simulink model "fft_direct_test"  (Simulink 7.2)
settings: Solver=VariableStepDiscrete  StartTime=0.0  StopTime=250  RelTol=1e-3
libraries: xbsIndex_r4 x249, casper_library_misc x24, simulink x1
(part 2 of 3)

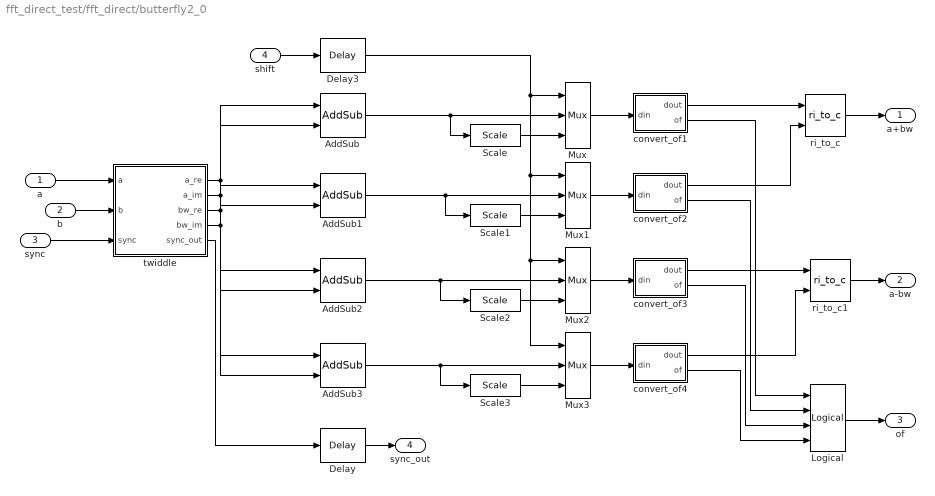
== system fft_direct_test/fft_direct/butterfly2_0 ==
  a : Inport  OutDataType=sfix(16)  OutScaling=2^0
  b : Inport  Port=2  OutDataType=sfix(16)  OutScaling=2^0
  sync : Inport  Port=3  OutDataType=sfix(16)  OutScaling=2^0
  shift : Inport  Port=4  OutDataType=sfix(16)  OutScaling=2^0
  AddSub : xbsIndex_r4/AddSub  mode=Addition  use_carryin=off  use_carryout=off  en=off  latency=add_latency  precision=Full  arith_type=Unsigned  n_bits=8  bin_pt=2  quantization=Truncate  overflow=Wrap  dbl_ovrd=off  use_behavioral_HDL=on  hw_selection=DSP48  pipelined=on  use_rpm=on  block_type=addsub
      settings: xl_area=[0, 0, 0, 0, 0, 0, 0]  block_version=9.1.01
  AddSub1 : xbsIndex_r4/AddSub  mode=Addition  use_carryin=off  use_carryout=off  en=off  latency=add_latency  precision=Full  arith_type=Unsigned  n_bits=8  bin_pt=2  quantization=Truncate  overflow=Wrap  dbl_ovrd=off  use_behavioral_HDL=on  hw_selection=DSP48  pipelined=on  use_rpm=on  block_type=addsub
      settings: xl_area=[0, 0, 0, 0, 0, 0, 0]  block_version=9.1.01
  AddSub2 : xbsIndex_r4/AddSub  mode=Subtraction  use_carryin=off  use_carryout=off  en=off  latency=add_latency  precision=Full  arith_type=Unsigned  n_bits=8  bin_pt=2  quantization=Truncate  overflow=Wrap  dbl_ovrd=off  use_behavioral_HDL=on  hw_selection=DSP48  pipelined=on  use_rpm=on  block_type=addsub
      settings: xl_area=[0, 0, 0, 0, 0, 0, 0]  block_version=9.1.01
  AddSub3 : xbsIndex_r4/AddSub  mode=Subtraction  use_carryin=off  use_carryout=off  en=off  latency=add_latency  precision=Full  arith_type=Unsigned  n_bits=8  bin_pt=2  quantization=Truncate  overflow=Wrap  dbl_ovrd=off  use_behavioral_HDL=on  hw_selection=DSP48  pipelined=on  use_rpm=on  block_type=addsub
      settings: xl_area=[0, 0, 0, 0, 0, 0, 0]  block_version=9.1.01
  Delay : xbsIndex_r4/Delay  en=off  latency=add_latency + conv_latency + 1  dbl_ovrd=off  reg_retiming=on  block_type=delay
      settings: xl_area=[0, 0, 0, 0, 0, 0, 0]  block_version=9.1.01
  Delay3 : xbsIndex_r4/Delay  en=off  latency=add_latency  dbl_ovrd=off  reg_retiming=off  block_type=delay
      settings: xl_area=[0, 0, 0, 0, 0, 0, 0]  block_version=9.1.01
  Logical : xbsIndex_r4/Logical  logical_function=OR  inputs=4  en=off  latency=0  precision=Full  arith_type=Unsigned  n_bits=16  bin_pt=0  align_bp=on  dbl_ovrd=off  block_type=logical
      settings: block_version=10.1.1
  Mux{,1..3} (4 alike) : xbsIndex_r4/Mux  inputs=2  en=off  latency=1  precision=Full  arith_type="Signed  (2's comp)"  n_bits=8  bin_pt=2  quantization=Truncate  overflow=Wrap  dbl_ovrd=off  block_type=mux
      settings: xl_area=[0, 0, 0, 0, 0, 0, 0]  block_version=9.1.01
  Scale{,1..3} (4 alike) : xbsIndex_r4/Scale  scale_factor=-1  dbl_ovrd=off  block_type=scale
      settings: infoedit=Scales input by a power of two by adjusting the binary point position.<P><P>Hardware notes: In hardware this block costs nothing.  block_version=9.1.01
  convert_of1 : Subsystem  AncestorBlock=casper_library_misc/convert_of  mask(convert_of){bit_width_i=14, binary_point_i=12, bit_width_o=12, binary_point_o=11, latency=2, overflow=Saturate, quantization=Truncate}
      mask prompts: bit_width_i "Bit Width In"; binary_point_i "Binary Point In"; bit_width_o "Bit Width Out"; binary_point_o "Binary Point Out"; overflow "Overflow Behaviour"; quantization "Quantization Behaviour"
      mask help:
      | Converts from one 2's complement bit-width
      | and/or binary point position to another.
      | Includes underflow/overflow indicator.
      mask init: same as fft_direct_test/fft_direct/butterfly1_0/convert_of1
      settings: AttributesFormatString=[14,12]->[12,11]
      mask StyleString: edit,edit,edit,edit,edit,popup(Wrap|Saturate|Error),popup(Truncate|Round  (unbiased: +/- Inf)|Round  (unbiased: even values))
  convert_of2 : Subsystem  AncestorBlock=casper_library_misc/convert_of  mask(convert_of){bit_width_i=14, binary_point_i=12, bit_width_o=12, binary_point_o=11, latency=2, overflow=Saturate, quantization=Truncate}
      mask prompts: bit_width_i "Bit Width In"; binary_point_i "Binary Point In"; bit_width_o "Bit Width Out"; binary_point_o "Binary Point Out"; overflow "Overflow Behaviour"; quantization "Quantization Behaviour"
      mask help:
      | Converts from one 2's complement bit-width
      | and/or binary point position to another.
      | Includes underflow/overflow indicator.
      mask init: same as fft_direct_test/fft_direct/butterfly1_0/convert_of1
      settings: AttributesFormatString=[14,12]->[12,11]
      mask StyleString: edit,edit,edit,edit,edit,popup(Wrap|Saturate|Error),popup(Truncate|Round  (unbiased: +/- Inf)|Round  (unbiased: even values))
  convert_of3 : Subsystem  AncestorBlock=casper_library_misc/convert_of  mask(convert_of){bit_width_i=14, binary_point_i=12, bit_width_o=12, binary_point_o=11, latency=2, overflow=Saturate, quantization=Truncate}
      mask prompts: bit_width_i "Bit Width In"; binary_point_i "Binary Point In"; bit_width_o "Bit Width Out"; binary_point_o "Binary Point Out"; overflow "Overflow Behaviour"; quantization "Quantization Behaviour"
      mask help:
      | Converts from one 2's complement bit-width
      | and/or binary point position to another.
      | Includes underflow/overflow indicator.
      mask init: same as fft_direct_test/fft_direct/butterfly1_0/convert_of1
      settings: AttributesFormatString=[14,12]->[12,11]
      mask StyleString: edit,edit,edit,edit,edit,popup(Wrap|Saturate|Error),popup(Truncate|Round  (unbiased: +/- Inf)|Round  (unbiased: even values))
  convert_of4 : Subsystem  AncestorBlock=casper_library_misc/convert_of  mask(convert_of){bit_width_i=14, binary_point_i=12, bit_width_o=12, binary_point_o=11, latency=2, overflow=Saturate, quantization=Truncate}
      mask prompts: bit_width_i "Bit Width In"; binary_point_i "Binary Point In"; bit_width_o "Bit Width Out"; binary_point_o "Binary Point Out"; overflow "Overflow Behaviour"; quantization "Quantization Behaviour"
      mask help:
      | Converts from one 2's complement bit-width
      | and/or binary point position to another.
      | Includes underflow/overflow indicator.
      mask init: same as fft_direct_test/fft_direct/butterfly1_0/convert_of1
      settings: AttributesFormatString=[14,12]->[12,11]
      mask StyleString: edit,edit,edit,edit,edit,popup(Wrap|Saturate|Error),popup(Truncate|Round  (unbiased: +/- Inf)|Round  (unbiased: even values))
  ri_to_c : casper_library_misc/ri_to_c  SystemSampleTime=-1
  ri_to_c1 : casper_library_misc/ri_to_c  SystemSampleTime=-1
  twiddle : Subsystem  AncestorBlock=casper_library_ffts_twiddle/twiddle_coeff_0  mask(twiddle_coeff_0){FFTSize=2, input_bit_width=12, add_latency=1, mult_latency=2, bram_latency=1, conv_latency=2, opt_target=multipliers}
      mask prompts: FFTSize "FFT Size (2^?)"; input_bit_width "Input Bit Width"; add_latency "Add Latency"; mult_latency "Mult Latency"; bram_latency "BRAM Latency"; conv_latency "Convert latency"; opt_target "Use less"
      mask help:
      | Used in FFT library. Used when coefficients
      | are 2^0 (just pass data through) but latency
      | must be the same as for a full twiddle.
      mask init: same as fft_direct_test/fft_direct/butterfly1_0/twiddle
      mask StyleString: edit,edit,edit,edit,edit,edit,popup(logic|multipliers)
  a+bw : Outport  OutDataType=sfix(16)  OutScaling=2^0
  a-bw : Outport  Port=2  OutDataType=sfix(16)  OutScaling=2^0
  of : Outport  Port=3  OutDataType=sfix(16)  OutScaling=2^0
  sync_out : Outport  Port=4  OutDataType=sfix(16)  OutScaling=2^0
  wires:
  convert_of4/2(of) -> Logical/4
  convert_of3/2(of) -> Logical/3
  convert_of2/2(of) -> Logical/2
  convert_of1/2(of) -> Logical/1
  convert_of4/1(dout) -> ri_to_c1/2
  Mux3/1 -> convert_of4/1(din)
  AddSub3/1 -> Scale3/1, Mux3/2
  Scale3/1 -> Mux3/3
  convert_of3/1(dout) -> ri_to_c1/1
  Mux2/1 -> convert_of3/1(din)
  AddSub2/1 -> Scale2/1, Mux2/2
  Scale2/1 -> Mux2/3
  convert_of2/1(dout) -> ri_to_c/2
  Mux1/1 -> convert_of2/1(din)
  AddSub1/1 -> Scale1/1, Mux1/2
  Scale1/1 -> Mux1/3
  convert_of1/1(dout) -> ri_to_c/1
  Mux/1 -> convert_of1/1(din)
  twiddle/4(bw_im) -> AddSub3/2, AddSub1/2
  twiddle/3(bw_re) -> AddSub2/2, AddSub/2
  twiddle/2(a_im) -> AddSub3/1, AddSub1/1
  twiddle/1(a_re) -> AddSub2/1, AddSub/1
  sync/1 -> twiddle/3(sync)
  b/1 -> twiddle/2(b)
  a/1 -> twiddle/1(a)
  ri_to_c/1 -> a+bw/1
  ri_to_c1/1 -> a-bw/1
  Delay/1 -> sync_out/1
  AddSub/1 -> Mux/2, Scale/1
  shift/1 -> Delay3/1
  Scale/1 -> Mux/3
  Delay3/1 -> Mux3/1, Mux2/1, Mux1/1, Mux/1
  Logical/1 -> of/1
  twiddle/5(sync_out) -> Delay/1

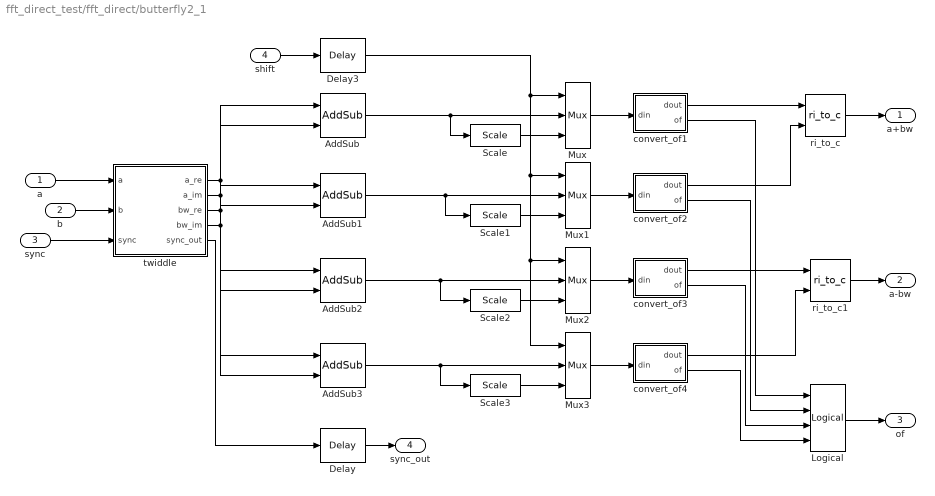
== system fft_direct_test/fft_direct/butterfly2_1 ==
  a : Inport  OutDataType=sfix(16)  OutScaling=2^0
  b : Inport  Port=2  OutDataType=sfix(16)  OutScaling=2^0
  sync : Inport  Port=3  OutDataType=sfix(16)  OutScaling=2^0
  shift : Inport  Port=4  OutDataType=sfix(16)  OutScaling=2^0
  AddSub : xbsIndex_r4/AddSub  mode=Addition  use_carryin=off  use_carryout=off  en=off  latency=add_latency  precision=Full  arith_type=Unsigned  n_bits=8  bin_pt=2  quantization=Truncate  overflow=Wrap  dbl_ovrd=off  use_behavioral_HDL=on  hw_selection=DSP48  pipelined=on  use_rpm=on  block_type=addsub
      settings: xl_area=[0, 0, 0, 0, 0, 0, 0]  block_version=9.1.01
  AddSub1 : xbsIndex_r4/AddSub  mode=Addition  use_carryin=off  use_carryout=off  en=off  latency=add_latency  precision=Full  arith_type=Unsigned  n_bits=8  bin_pt=2  quantization=Truncate  overflow=Wrap  dbl_ovrd=off  use_behavioral_HDL=on  hw_selection=DSP48  pipelined=on  use_rpm=on  block_type=addsub
      settings: xl_area=[0, 0, 0, 0, 0, 0, 0]  block_version=9.1.01
  AddSub2 : xbsIndex_r4/AddSub  mode=Subtraction  use_carryin=off  use_carryout=off  en=off  latency=add_latency  precision=Full  arith_type=Unsigned  n_bits=8  bin_pt=2  quantization=Truncate  overflow=Wrap  dbl_ovrd=off  use_behavioral_HDL=on  hw_selection=DSP48  pipelined=on  use_rpm=on  block_type=addsub
      settings: xl_area=[0, 0, 0, 0, 0, 0, 0]  block_version=9.1.01
  AddSub3 : xbsIndex_r4/AddSub  mode=Subtraction  use_carryin=off  use_carryout=off  en=off  latency=add_latency  precision=Full  arith_type=Unsigned  n_bits=8  bin_pt=2  quantization=Truncate  overflow=Wrap  dbl_ovrd=off  use_behavioral_HDL=on  hw_selection=DSP48  pipelined=on  use_rpm=on  block_type=addsub
      settings: xl_area=[0, 0, 0, 0, 0, 0, 0]  block_version=9.1.01
  Delay : xbsIndex_r4/Delay  en=off  latency=add_latency + conv_latency + 1  dbl_ovrd=off  reg_retiming=on  block_type=delay
      settings: xl_area=[0, 0, 0, 0, 0, 0, 0]  block_version=9.1.01
  Delay3 : xbsIndex_r4/Delay  en=off  latency=add_latency  dbl_ovrd=off  reg_retiming=off  block_type=delay
      settings: xl_area=[0, 0, 0, 0, 0, 0, 0]  block_version=9.1.01
  Logical : xbsIndex_r4/Logical  logical_function=OR  inputs=4  en=off  latency=0  precision=Full  arith_type=Unsigned  n_bits=16  bin_pt=0  align_bp=on  dbl_ovrd=off  block_type=logical
      settings: block_version=10.1.1
  Mux{,1..3} (4 alike) : xbsIndex_r4/Mux  inputs=2  en=off  latency=1  precision=Full  arith_type="Signed  (2's comp)"  n_bits=8  bin_pt=2  quantization=Truncate  overflow=Wrap  dbl_ovrd=off  block_type=mux
      settings: xl_area=[0, 0, 0, 0, 0, 0, 0]  block_version=9.1.01
  Scale{,1..3} (4 alike) : xbsIndex_r4/Scale  scale_factor=-1  dbl_ovrd=off  block_type=scale
      settings: infoedit=Scales input by a power of two by adjusting the binary point position.<P><P>Hardware notes: In hardware this block costs nothing.  block_version=9.1.01
  convert_of1 : Subsystem  AncestorBlock=casper_library_misc/convert_of  mask(convert_of){bit_width_i=14, binary_point_i=12, bit_width_o=12, binary_point_o=11, latency=2, overflow=Saturate, quantization=Truncate}
      mask prompts: bit_width_i "Bit Width In"; binary_point_i "Binary Point In"; bit_width_o "Bit Width Out"; binary_point_o "Binary Point Out"; overflow "Overflow Behaviour"; quantization "Quantization Behaviour"
      mask help:
      | Converts from one 2's complement bit-width
      | and/or binary point position to another.
      | Includes underflow/overflow indicator.
      mask init: same as fft_direct_test/fft_direct/butterfly1_0/convert_of1
      settings: AttributesFormatString=[14,12]->[12,11]
      mask StyleString: edit,edit,edit,edit,edit,popup(Wrap|Saturate|Error),popup(Truncate|Round  (unbiased: +/- Inf)|Round  (unbiased: even values))
  convert_of2 : Subsystem  AncestorBlock=casper_library_misc/convert_of  mask(convert_of){bit_width_i=14, binary_point_i=12, bit_width_o=12, binary_point_o=11, latency=2, overflow=Saturate, quantization=Truncate}
      mask prompts: bit_width_i "Bit Width In"; binary_point_i "Binary Point In"; bit_width_o "Bit Width Out"; binary_point_o "Binary Point Out"; overflow "Overflow Behaviour"; quantization "Quantization Behaviour"
      mask help:
      | Converts from one 2's complement bit-width
      | and/or binary point position to another.
      | Includes underflow/overflow indicator.
      mask init: same as fft_direct_test/fft_direct/butterfly1_0/convert_of1
      settings: AttributesFormatString=[14,12]->[12,11]
      mask StyleString: edit,edit,edit,edit,edit,popup(Wrap|Saturate|Error),popup(Truncate|Round  (unbiased: +/- Inf)|Round  (unbiased: even values))
  convert_of3 : Subsystem  AncestorBlock=casper_library_misc/convert_of  mask(convert_of){bit_width_i=14, binary_point_i=12, bit_width_o=12, binary_point_o=11, latency=2, overflow=Saturate, quantization=Truncate}
      mask prompts: bit_width_i "Bit Width In"; binary_point_i "Binary Point In"; bit_width_o "Bit Width Out"; binary_point_o "Binary Point Out"; overflow "Overflow Behaviour"; quantization "Quantization Behaviour"
      mask help:
      | Converts from one 2's complement bit-width
      | and/or binary point position to another.
      | Includes underflow/overflow indicator.
      mask init: same as fft_direct_test/fft_direct/butterfly1_0/convert_of1
      settings: AttributesFormatString=[14,12]->[12,11]
      mask StyleString: edit,edit,edit,edit,edit,popup(Wrap|Saturate|Error),popup(Truncate|Round  (unbiased: +/- Inf)|Round  (unbiased: even values))
  convert_of4 : Subsystem  AncestorBlock=casper_library_misc/convert_of  mask(convert_of){bit_width_i=14, binary_point_i=12, bit_width_o=12, binary_point_o=11, latency=2, overflow=Saturate, quantization=Truncate}
      mask prompts: bit_width_i "Bit Width In"; binary_point_i "Binary Point In"; bit_width_o "Bit Width Out"; binary_point_o "Binary Point Out"; overflow "Overflow Behaviour"; quantization "Quantization Behaviour"
      mask help:
      | Converts from one 2's complement bit-width
      | and/or binary point position to another.
      | Includes underflow/overflow indicator.
      mask init: same as fft_direct_test/fft_direct/butterfly1_0/convert_of1
      settings: AttributesFormatString=[14,12]->[12,11]
      mask StyleString: edit,edit,edit,edit,edit,popup(Wrap|Saturate|Error),popup(Truncate|Round  (unbiased: +/- Inf)|Round  (unbiased: even values))
  ri_to_c : casper_library_misc/ri_to_c  SystemSampleTime=-1
  ri_to_c1 : casper_library_misc/ri_to_c  SystemSampleTime=-1
  twiddle : Subsystem  AncestorBlock=casper_library_ffts_twiddle/twiddle_coeff_1  mask(twiddle_coeff_1){FFTSize=2, input_bit_width=12, add_latency=1, mult_latency=2, bram_latency=1, conv_latency=2, opt_target=multipliers}
      mask prompts: FFTSize "FFT Size (2^?)"; input_bit_width "Input Bit Width"; add_latency "Add Latency"; mult_latency "Mult Latency"; bram_latency "BRAM Latency"; conv_latency "Convert latency"; opt_target "Use less"
      mask help:
      | Used in FFT library. Used when result of
      | coeff*(a+jb)=b-ja
      mask init:
      | set_param(gcb,'LinkStatus','inactive');
      | if(strcmp(opt_target, 'logic')), 
      |     latency = 'mult_latency+add_latency+bram_latency+conv_latency';
      | else,
      |     latency = 'mult_latency+add_latency*2+bram_latency+conv_latency';
      | end
      | set_param([gcb,'/delay0'], 'latency', latency);
      | set_param([gcb,'/delay1'], 'latency', latency);
      | set_param([gcb,'/delay2'], 'latency', latency);
      | set_param([gcb,'/delay3'], 'latency', latency);
      | set_param([gcb,'/negate'], 'latency', latency);
      mask StyleString: edit,edit,edit,edit,edit,edit,popup(logic|multipliers)
  a+bw : Outport  OutDataType=sfix(16)  OutScaling=2^0
  a-bw : Outport  Port=2  OutDataType=sfix(16)  OutScaling=2^0
  of : Outport  Port=3  OutDataType=sfix(16)  OutScaling=2^0
  sync_out : Outport  Port=4  OutDataType=sfix(16)  OutScaling=2^0
  wires:
  convert_of4/2(of) -> Logical/4
  convert_of3/2(of) -> Logical/3
  convert_of2/2(of) -> Logical/2
  convert_of1/2(of) -> Logical/1
  convert_of4/1(dout) -> ri_to_c1/2
  Mux3/1 -> convert_of4/1(din)
  AddSub3/1 -> Scale3/1, Mux3/2
  Scale3/1 -> Mux3/3
  convert_of3/1(dout) -> ri_to_c1/1
  Mux2/1 -> convert_of3/1(din)
  AddSub2/1 -> Scale2/1, Mux2/2
  Scale2/1 -> Mux2/3
  convert_of2/1(dout) -> ri_to_c/2
  Mux1/1 -> convert_of2/1(din)
  AddSub1/1 -> Scale1/1, Mux1/2
  Scale1/1 -> Mux1/3
  convert_of1/1(dout) -> ri_to_c/1
  Mux/1 -> convert_of1/1(din)
  twiddle/4(bw_im) -> AddSub3/2, AddSub1/2
  twiddle/3(bw_re) -> AddSub2/2, AddSub/2
  twiddle/2(a_im) -> AddSub3/1, AddSub1/1
  twiddle/1(a_re) -> AddSub2/1, AddSub/1
  sync/1 -> twiddle/3(sync)
  b/1 -> twiddle/2(b)
  a/1 -> twiddle/1(a)
  ri_to_c/1 -> a+bw/1
  ri_to_c1/1 -> a-bw/1
  Delay/1 -> sync_out/1
  AddSub/1 -> Mux/2, Scale/1
  shift/1 -> Delay3/1
  Scale/1 -> Mux/3
  Delay3/1 -> Mux3/1, Mux2/1, Mux1/1, Mux/1
  Logical/1 -> of/1
  twiddle/5(sync_out) -> Delay/1

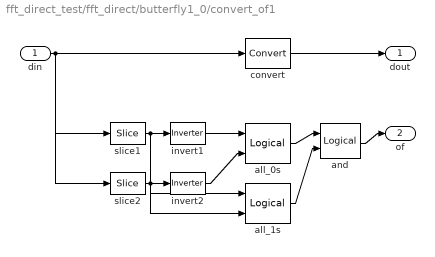
== system fft_direct_test/fft_direct/butterfly1_0/convert_of1 ==
  din : Inport  OutDataType=sfix(16)  OutScaling=2^0
  all_0s : xbsIndex_r4/Logical  logical_function=NAND  inputs=2  en=off  latency=latency  precision=Full  arith_type=Unsigned  n_bits=16  bin_pt=0  align_bp=on  dbl_ovrd=off  block_type=logical
  all_1s : xbsIndex_r4/Logical  logical_function=NAND  inputs=2  en=off  latency=latency  precision=Full  arith_type=Unsigned  n_bits=16  bin_pt=0  align_bp=on  dbl_ovrd=off  block_type=logical
  and : xbsIndex_r4/Logical  logical_function=AND  inputs=2  en=off  latency=0  precision=Full  arith_type=Unsigned  n_bits=16  bin_pt=0  align_bp=on  dbl_ovrd=off  block_type=logical
  convert : xbsIndex_r4/Convert  arith_type="Signed  (2's comp)"  n_bits=bit_width_o  bin_pt=binary_point_o  quantization=Truncate  overflow=Saturate  latency=latency  dbl_ovrd=off  pipeline=on  block_type=convert
      settings: block_version=10.1.1
  invert1 : xbsIndex_r4/Inverter  en=off  latency=0  dbl_ovrd=off  block_type=inv
  invert2 : xbsIndex_r4/Inverter  en=off  latency=0  dbl_ovrd=off  block_type=inv
  slice1 : xbsIndex_r4/Slice  nbits=1  boolean_output=on  mode=Upper Bit Location + Width  bit1=0  base1=MSB of Input  bit0=0  base0=LSB of Input  dbl_ovrd=off  block_type=slice
      settings: infoedit="Extracts a given range of bits from each input sample and presents it at the output.  The output type is ordinarily unsigned with binary point at zero, but can be Boolean when the slice is one bit wide.<P><P>Hardware notes: In hardware this block costs nothing."  block_version=10.1.1
  slice2 : xbsIndex_r4/Slice  nbits=1  boolean_output=on  mode=Upper Bit Location + Width  bit1=-1  base1=MSB of Input  bit0=0  base0=LSB of Input  dbl_ovrd=off  block_type=slice
      settings: infoedit="Extracts a given range of bits from each input sample and presents it at the output.  The output type is ordinarily unsigned with binary point at zero, but can be Boolean when the slice is one bit wide.<P><P>Hardware notes: In hardware this block costs nothing."  block_version=10.1.1
  dout : Outport
  of : Outport  Port=2
  wires:
  din/1 -> convert/1, slice1/1, slice2/1
  convert/1 -> dout/1
  slice1/1 -> all_1s/1, invert1/1
  invert1/1 -> all_0s/1
  slice2/1 -> all_1s/2, invert2/1
  invert2/1 -> all_0s/2
  all_0s/1 -> and/1
  all_1s/1 -> and/2
  and/1 -> of/1

== system fft_direct_test/fft_direct/butterfly1_0/convert_of2 ==
  din : Inport  OutDataType=sfix(16)  OutScaling=2^0
  all_0s : xbsIndex_r4/Logical  logical_function=NAND  inputs=2  en=off  latency=latency  precision=Full  arith_type=Unsigned  n_bits=16  bin_pt=0  align_bp=on  dbl_ovrd=off  block_type=logical
  all_1s : xbsIndex_r4/Logical  logical_function=NAND  inputs=2  en=off  latency=latency  precision=Full  arith_type=Unsigned  n_bits=16  bin_pt=0  align_bp=on  dbl_ovrd=off  block_type=logical
  and : xbsIndex_r4/Logical  logical_function=AND  inputs=2  en=off  latency=0  precision=Full  arith_type=Unsigned  n_bits=16  bin_pt=0  align_bp=on  dbl_ovrd=off  block_type=logical
  convert : xbsIndex_r4/Convert  arith_type="Signed  (2's comp)"  n_bits=bit_width_o  bin_pt=binary_point_o  quantization=Truncate  overflow=Saturate  latency=latency  dbl_ovrd=off  pipeline=on  block_type=convert
      settings: block_version=10.1.1
  invert1 : xbsIndex_r4/Inverter  en=off  latency=0  dbl_ovrd=off  block_type=inv
  invert2 : xbsIndex_r4/Inverter  en=off  latency=0  dbl_ovrd=off  block_type=inv
  slice1 : xbsIndex_r4/Slice  nbits=1  boolean_output=on  mode=Upper Bit Location + Width  bit1=0  base1=MSB of Input  bit0=0  base0=LSB of Input  dbl_ovrd=off  block_type=slice
      settings: infoedit="Extracts a given range of bits from each input sample and presents it at the output.  The output type is ordinarily unsigned with binary point at zero, but can be Boolean when the slice is one bit wide.<P><P>Hardware notes: In hardware this block costs nothing."  block_version=10.1.1
  slice2 : xbsIndex_r4/Slice  nbits=1  boolean_output=on  mode=Upper Bit Location + Width  bit1=-1  base1=MSB of Input  bit0=0  base0=LSB of Input  dbl_ovrd=off  block_type=slice
      settings: infoedit="Extracts a given range of bits from each input sample and presents it at the output.  The output type is ordinarily unsigned with binary point at zero, but can be Boolean when the slice is one bit wide.<P><P>Hardware notes: In hardware this block costs nothing."  block_version=10.1.1
  dout : Outport
  of : Outport  Port=2
  wires:
  din/1 -> convert/1, slice1/1, slice2/1
  convert/1 -> dout/1
  slice1/1 -> all_1s/1, invert1/1
  invert1/1 -> all_0s/1
  slice2/1 -> all_1s/2, invert2/1
  invert2/1 -> all_0s/2
  all_0s/1 -> and/1
  all_1s/1 -> and/2
  and/1 -> of/1

== system fft_direct_test/fft_direct/butterfly1_0/convert_of3 ==
  din : Inport  OutDataType=sfix(16)  OutScaling=2^0
  all_0s : xbsIndex_r4/Logical  logical_function=NAND  inputs=2  en=off  latency=latency  precision=Full  arith_type=Unsigned  n_bits=16  bin_pt=0  align_bp=on  dbl_ovrd=off  block_type=logical
  all_1s : xbsIndex_r4/Logical  logical_function=NAND  inputs=2  en=off  latency=latency  precision=Full  arith_type=Unsigned  n_bits=16  bin_pt=0  align_bp=on  dbl_ovrd=off  block_type=logical
  and : xbsIndex_r4/Logical  logical_function=AND  inputs=2  en=off  latency=0  precision=Full  arith_type=Unsigned  n_bits=16  bin_pt=0  align_bp=on  dbl_ovrd=off  block_type=logical
  convert : xbsIndex_r4/Convert  arith_type="Signed  (2's comp)"  n_bits=bit_width_o  bin_pt=binary_point_o  quantization=Truncate  overflow=Saturate  latency=latency  dbl_ovrd=off  pipeline=on  block_type=convert
      settings: block_version=10.1.1
  invert1 : xbsIndex_r4/Inverter  en=off  latency=0  dbl_ovrd=off  block_type=inv
  invert2 : xbsIndex_r4/Inverter  en=off  latency=0  dbl_ovrd=off  block_type=inv
  slice1 : xbsIndex_r4/Slice  nbits=1  boolean_output=on  mode=Upper Bit Location + Width  bit1=0  base1=MSB of Input  bit0=0  base0=LSB of Input  dbl_ovrd=off  block_type=slice
      settings: infoedit="Extracts a given range of bits from each input sample and presents it at the output.  The output type is ordinarily unsigned with binary point at zero, but can be Boolean when the slice is one bit wide.<P><P>Hardware notes: In hardware this block costs nothing."  block_version=10.1.1
  slice2 : xbsIndex_r4/Slice  nbits=1  boolean_output=on  mode=Upper Bit Location + Width  bit1=-1  base1=MSB of Input  bit0=0  base0=LSB of Input  dbl_ovrd=off  block_type=slice
      settings: infoedit="Extracts a given range of bits from each input sample and presents it at the output.  The output type is ordinarily unsigned with binary point at zero, but can be Boolean when the slice is one bit wide.<P><P>Hardware notes: In hardware this block costs nothing."  block_version=10.1.1
  dout : Outport
  of : Outport  Port=2
  wires:
  din/1 -> convert/1, slice1/1, slice2/1
  convert/1 -> dout/1
  slice1/1 -> all_1s/1, invert1/1
  invert1/1 -> all_0s/1
  slice2/1 -> all_1s/2, invert2/1
  invert2/1 -> all_0s/2
  all_0s/1 -> and/1
  all_1s/1 -> and/2
  and/1 -> of/1

== system fft_direct_test/fft_direct/butterfly1_0/convert_of4 ==
  din : Inport  OutDataType=sfix(16)  OutScaling=2^0
  all_0s : xbsIndex_r4/Logical  logical_function=NAND  inputs=2  en=off  latency=latency  precision=Full  arith_type=Unsigned  n_bits=16  bin_pt=0  align_bp=on  dbl_ovrd=off  block_type=logical
  all_1s : xbsIndex_r4/Logical  logical_function=NAND  inputs=2  en=off  latency=latency  precision=Full  arith_type=Unsigned  n_bits=16  bin_pt=0  align_bp=on  dbl_ovrd=off  block_type=logical
  and : xbsIndex_r4/Logical  logical_function=AND  inputs=2  en=off  latency=0  precision=Full  arith_type=Unsigned  n_bits=16  bin_pt=0  align_bp=on  dbl_ovrd=off  block_type=logical
  convert : xbsIndex_r4/Convert  arith_type="Signed  (2's comp)"  n_bits=bit_width_o  bin_pt=binary_point_o  quantization=Truncate  overflow=Saturate  latency=latency  dbl_ovrd=off  pipeline=on  block_type=convert
      settings: block_version=10.1.1
  invert1 : xbsIndex_r4/Inverter  en=off  latency=0  dbl_ovrd=off  block_type=inv
  invert2 : xbsIndex_r4/Inverter  en=off  latency=0  dbl_ovrd=off  block_type=inv
  slice1 : xbsIndex_r4/Slice  nbits=1  boolean_output=on  mode=Upper Bit Location + Width  bit1=0  base1=MSB of Input  bit0=0  base0=LSB of Input  dbl_ovrd=off  block_type=slice
      settings: infoedit="Extracts a given range of bits from each input sample and presents it at the output.  The output type is ordinarily unsigned with binary point at zero, but can be Boolean when the slice is one bit wide.<P><P>Hardware notes: In hardware this block costs nothing."  block_version=10.1.1
  slice2 : xbsIndex_r4/Slice  nbits=1  boolean_output=on  mode=Upper Bit Location + Width  bit1=-1  base1=MSB of Input  bit0=0  base0=LSB of Input  dbl_ovrd=off  block_type=slice
      settings: infoedit="Extracts a given range of bits from each input sample and presents it at the output.  The output type is ordinarily unsigned with binary point at zero, but can be Boolean when the slice is one bit wide.<P><P>Hardware notes: In hardware this block costs nothing."  block_version=10.1.1
  dout : Outport
  of : Outport  Port=2
  wires:
  din/1 -> convert/1, slice1/1, slice2/1
  convert/1 -> dout/1
  slice1/1 -> all_1s/1, invert1/1
  invert1/1 -> all_0s/1
  slice2/1 -> all_1s/2, invert2/1
  invert2/1 -> all_0s/2
  all_0s/1 -> and/1
  all_1s/1 -> and/2
  and/1 -> of/1

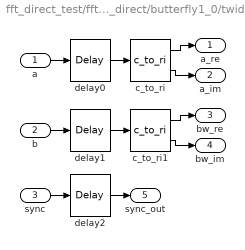
== system fft_direct_test/fft_direct/butterfly1_0/twiddle ==
  a : Inport  OutDataType=sfix(16)  OutScaling=2^0
  b : Inport  Port=2  OutDataType=sfix(16)  OutScaling=2^0
  sync : Inport  Port=3  OutDataType=sfix(16)  OutScaling=2^0
  c_to_ri : casper_library_misc/c_to_ri  SystemSampleTime=-1  n_bits=input_bit_width  bin_pt=input_bit_width-1
      settings: AttributesFormatString=12_11 r/i
  c_to_ri1 : casper_library_misc/c_to_ri  SystemSampleTime=-1  n_bits=input_bit_width  bin_pt=input_bit_width-1
      settings: AttributesFormatString=12_11 r/i
  delay0 : xbsIndex_r4/Delay  en=off  latency=mult_latency+add_latency*2+bram_latency+conv_latency  dbl_ovrd=off  reg_retiming=on  block_type=delay
  delay1 : xbsIndex_r4/Delay  en=off  latency=mult_latency+add_latency*2+bram_latency+conv_latency  dbl_ovrd=off  reg_retiming=on  block_type=delay
  delay2 : xbsIndex_r4/Delay  en=off  latency=mult_latency+add_latency*2+bram_latency+conv_latency  dbl_ovrd=off  reg_retiming=on  block_type=delay
  a_re : Outport  OutDataType=sfix(16)  OutScaling=2^0
  a_im : Outport  Port=2  OutDataType=sfix(16)  OutScaling=2^0
  bw_re : Outport  Port=3  OutDataType=sfix(16)  OutScaling=2^0
  bw_im : Outport  Port=4  OutDataType=sfix(16)  OutScaling=2^0
  sync_out : Outport  Port=5  OutDataType=sfix(16)  OutScaling=2^0
  wires:
  delay2/1 -> sync_out/1
  delay1/1 -> c_to_ri1/1
  delay0/1 -> c_to_ri/1
  a/1 -> delay0/1
  sync/1 -> delay2/1
  b/1 -> delay1/1
  c_to_ri/1 -> a_re/1
  c_to_ri/2 -> a_im/1
  c_to_ri1/1 -> bw_re/1
  c_to_ri1/2 -> bw_im/1

== system fft_direct_test/fft_direct/butterfly1_1/convert_of1 ==
  din : Inport  OutDataType=sfix(16)  OutScaling=2^0
  all_0s : xbsIndex_r4/Logical  logical_function=NAND  inputs=2  en=off  latency=latency  precision=Full  arith_type=Unsigned  n_bits=16  bin_pt=0  align_bp=on  dbl_ovrd=off  block_type=logical
  all_1s : xbsIndex_r4/Logical  logical_function=NAND  inputs=2  en=off  latency=latency  precision=Full  arith_type=Unsigned  n_bits=16  bin_pt=0  align_bp=on  dbl_ovrd=off  block_type=logical
  and : xbsIndex_r4/Logical  logical_function=AND  inputs=2  en=off  latency=0  precision=Full  arith_type=Unsigned  n_bits=16  bin_pt=0  align_bp=on  dbl_ovrd=off  block_type=logical
  convert : xbsIndex_r4/Convert  arith_type="Signed  (2's comp)"  n_bits=bit_width_o  bin_pt=binary_point_o  quantization=Truncate  overflow=Saturate  latency=latency  dbl_ovrd=off  pipeline=on  block_type=convert
      settings: block_version=10.1.1
  invert1 : xbsIndex_r4/Inverter  en=off  latency=0  dbl_ovrd=off  block_type=inv
  invert2 : xbsIndex_r4/Inverter  en=off  latency=0  dbl_ovrd=off  block_type=inv
  slice1 : xbsIndex_r4/Slice  nbits=1  boolean_output=on  mode=Upper Bit Location + Width  bit1=0  base1=MSB of Input  bit0=0  base0=LSB of Input  dbl_ovrd=off  block_type=slice
      settings: infoedit="Extracts a given range of bits from each input sample and presents it at the output.  The output type is ordinarily unsigned with binary point at zero, but can be Boolean when the slice is one bit wide.<P><P>Hardware notes: In hardware this block costs nothing."  block_version=10.1.1
  slice2 : xbsIndex_r4/Slice  nbits=1  boolean_output=on  mode=Upper Bit Location + Width  bit1=-1  base1=MSB of Input  bit0=0  base0=LSB of Input  dbl_ovrd=off  block_type=slice
      settings: infoedit="Extracts a given range of bits from each input sample and presents it at the output.  The output type is ordinarily unsigned with binary point at zero, but can be Boolean when the slice is one bit wide.<P><P>Hardware notes: In hardware this block costs nothing."  block_version=10.1.1
  dout : Outport
  of : Outport  Port=2
  wires:
  din/1 -> convert/1, slice1/1, slice2/1
  convert/1 -> dout/1
  slice1/1 -> all_1s/1, invert1/1
  invert1/1 -> all_0s/1
  slice2/1 -> all_1s/2, invert2/1
  invert2/1 -> all_0s/2
  all_0s/1 -> and/1
  all_1s/1 -> and/2
  and/1 -> of/1

== system fft_direct_test/fft_direct/butterfly1_1/convert_of2 ==
  din : Inport  OutDataType=sfix(16)  OutScaling=2^0
  all_0s : xbsIndex_r4/Logical  logical_function=NAND  inputs=2  en=off  latency=latency  precision=Full  arith_type=Unsigned  n_bits=16  bin_pt=0  align_bp=on  dbl_ovrd=off  block_type=logical
  all_1s : xbsIndex_r4/Logical  logical_function=NAND  inputs=2  en=off  latency=latency  precision=Full  arith_type=Unsigned  n_bits=16  bin_pt=0  align_bp=on  dbl_ovrd=off  block_type=logical
  and : xbsIndex_r4/Logical  logical_function=AND  inputs=2  en=off  latency=0  precision=Full  arith_type=Unsigned  n_bits=16  bin_pt=0  align_bp=on  dbl_ovrd=off  block_type=logical
  convert : xbsIndex_r4/Convert  arith_type="Signed  (2's comp)"  n_bits=bit_width_o  bin_pt=binary_point_o  quantization=Truncate  overflow=Saturate  latency=latency  dbl_ovrd=off  pipeline=on  block_type=convert
      settings: block_version=10.1.1
  invert1 : xbsIndex_r4/Inverter  en=off  latency=0  dbl_ovrd=off  block_type=inv
  invert2 : xbsIndex_r4/Inverter  en=off  latency=0  dbl_ovrd=off  block_type=inv
  slice1 : xbsIndex_r4/Slice  nbits=1  boolean_output=on  mode=Upper Bit Location + Width  bit1=0  base1=MSB of Input  bit0=0  base0=LSB of Input  dbl_ovrd=off  block_type=slice
      settings: infoedit="Extracts a given range of bits from each input sample and presents it at the output.  The output type is ordinarily unsigned with binary point at zero, but can be Boolean when the slice is one bit wide.<P><P>Hardware notes: In hardware this block costs nothing."  block_version=10.1.1
  slice2 : xbsIndex_r4/Slice  nbits=1  boolean_output=on  mode=Upper Bit Location + Width  bit1=-1  base1=MSB of Input  bit0=0  base0=LSB of Input  dbl_ovrd=off  block_type=slice
      settings: infoedit="Extracts a given range of bits from each input sample and presents it at the output.  The output type is ordinarily unsigned with binary point at zero, but can be Boolean when the slice is one bit wide.<P><P>Hardware notes: In hardware this block costs nothing."  block_version=10.1.1
  dout : Outport
  of : Outport  Port=2
  wires:
  din/1 -> convert/1, slice1/1, slice2/1
  convert/1 -> dout/1
  slice1/1 -> all_1s/1, invert1/1
  invert1/1 -> all_0s/1
  slice2/1 -> all_1s/2, invert2/1
  invert2/1 -> all_0s/2
  all_0s/1 -> and/1
  all_1s/1 -> and/2
  and/1 -> of/1

== system fft_direct_test/fft_direct/butterfly1_1/convert_of3 ==
  din : Inport  OutDataType=sfix(16)  OutScaling=2^0
  all_0s : xbsIndex_r4/Logical  logical_function=NAND  inputs=2  en=off  latency=latency  precision=Full  arith_type=Unsigned  n_bits=16  bin_pt=0  align_bp=on  dbl_ovrd=off  block_type=logical
  all_1s : xbsIndex_r4/Logical  logical_function=NAND  inputs=2  en=off  latency=latency  precision=Full  arith_type=Unsigned  n_bits=16  bin_pt=0  align_bp=on  dbl_ovrd=off  block_type=logical
  and : xbsIndex_r4/Logical  logical_function=AND  inputs=2  en=off  latency=0  precision=Full  arith_type=Unsigned  n_bits=16  bin_pt=0  align_bp=on  dbl_ovrd=off  block_type=logical
  convert : xbsIndex_r4/Convert  arith_type="Signed  (2's comp)"  n_bits=bit_width_o  bin_pt=binary_point_o  quantization=Truncate  overflow=Saturate  latency=latency  dbl_ovrd=off  pipeline=on  block_type=convert
      settings: block_version=10.1.1
  invert1 : xbsIndex_r4/Inverter  en=off  latency=0  dbl_ovrd=off  block_type=inv
  invert2 : xbsIndex_r4/Inverter  en=off  latency=0  dbl_ovrd=off  block_type=inv
  slice1 : xbsIndex_r4/Slice  nbits=1  boolean_output=on  mode=Upper Bit Location + Width  bit1=0  base1=MSB of Input  bit0=0  base0=LSB of Input  dbl_ovrd=off  block_type=slice
      settings: infoedit="Extracts a given range of bits from each input sample and presents it at the output.  The output type is ordinarily unsigned with binary point at zero, but can be Boolean when the slice is one bit wide.<P><P>Hardware notes: In hardware this block costs nothing."  block_version=10.1.1
  slice2 : xbsIndex_r4/Slice  nbits=1  boolean_output=on  mode=Upper Bit Location + Width  bit1=-1  base1=MSB of Input  bit0=0  base0=LSB of Input  dbl_ovrd=off  block_type=slice
      settings: infoedit="Extracts a given range of bits from each input sample and presents it at the output.  The output type is ordinarily unsigned with binary point at zero, but can be Boolean when the slice is one bit wide.<P><P>Hardware notes: In hardware this block costs nothing."  block_version=10.1.1
  dout : Outport
  of : Outport  Port=2
  wires:
  din/1 -> convert/1, slice1/1, slice2/1
  convert/1 -> dout/1
  slice1/1 -> all_1s/1, invert1/1
  invert1/1 -> all_0s/1
  slice2/1 -> all_1s/2, invert2/1
  invert2/1 -> all_0s/2
  all_0s/1 -> and/1
  all_1s/1 -> and/2
  and/1 -> of/1

== system fft_direct_test/fft_direct/butterfly1_1/convert_of4 ==
  din : Inport  OutDataType=sfix(16)  OutScaling=2^0
  all_0s : xbsIndex_r4/Logical  logical_function=NAND  inputs=2  en=off  latency=latency  precision=Full  arith_type=Unsigned  n_bits=16  bin_pt=0  align_bp=on  dbl_ovrd=off  block_type=logical
  all_1s : xbsIndex_r4/Logical  logical_function=NAND  inputs=2  en=off  latency=latency  precision=Full  arith_type=Unsigned  n_bits=16  bin_pt=0  align_bp=on  dbl_ovrd=off  block_type=logical
  and : xbsIndex_r4/Logical  logical_function=AND  inputs=2  en=off  latency=0  precision=Full  arith_type=Unsigned  n_bits=16  bin_pt=0  align_bp=on  dbl_ovrd=off  block_type=logical
  convert : xbsIndex_r4/Convert  arith_type="Signed  (2's comp)"  n_bits=bit_width_o  bin_pt=binary_point_o  quantization=Truncate  overflow=Saturate  latency=latency  dbl_ovrd=off  pipeline=on  block_type=convert
      settings: block_version=10.1.1
  invert1 : xbsIndex_r4/Inverter  en=off  latency=0  dbl_ovrd=off  block_type=inv
  invert2 : xbsIndex_r4/Inverter  en=off  latency=0  dbl_ovrd=off  block_type=inv
  slice1 : xbsIndex_r4/Slice  nbits=1  boolean_output=on  mode=Upper Bit Location + Width  bit1=0  base1=MSB of Input  bit0=0  base0=LSB of Input  dbl_ovrd=off  block_type=slice
      settings: infoedit="Extracts a given range of bits from each input sample and presents it at the output.  The output type is ordinarily unsigned with binary point at zero, but can be Boolean when the slice is one bit wide.<P><P>Hardware notes: In hardware this block costs nothing."  block_version=10.1.1
  slice2 : xbsIndex_r4/Slice  nbits=1  boolean_output=on  mode=Upper Bit Location + Width  bit1=-1  base1=MSB of Input  bit0=0  base0=LSB of Input  dbl_ovrd=off  block_type=slice
      settings: infoedit="Extracts a given range of bits from each input sample and presents it at the output.  The output type is ordinarily unsigned with binary point at zero, but can be Boolean when the slice is one bit wide.<P><P>Hardware notes: In hardware this block costs nothing."  block_version=10.1.1
  dout : Outport
  of : Outport  Port=2
  wires:
  din/1 -> convert/1, slice1/1, slice2/1
  convert/1 -> dout/1
  slice1/1 -> all_1s/1, invert1/1
  invert1/1 -> all_0s/1
  slice2/1 -> all_1s/2, invert2/1
  invert2/1 -> all_0s/2
  all_0s/1 -> and/1
  all_1s/1 -> and/2
  and/1 -> of/1

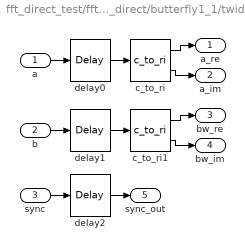
== system fft_direct_test/fft_direct/butterfly1_1/twiddle ==
  a : Inport  OutDataType=sfix(16)  OutScaling=2^0
  b : Inport  Port=2  OutDataType=sfix(16)  OutScaling=2^0
  sync : Inport  Port=3  OutDataType=sfix(16)  OutScaling=2^0
  c_to_ri : casper_library_misc/c_to_ri  SystemSampleTime=-1  n_bits=input_bit_width  bin_pt=input_bit_width-1
      settings: AttributesFormatString=12_11 r/i
  c_to_ri1 : casper_library_misc/c_to_ri  SystemSampleTime=-1  n_bits=input_bit_width  bin_pt=input_bit_width-1
      settings: AttributesFormatString=12_11 r/i
  delay0 : xbsIndex_r4/Delay  en=off  latency=mult_latency+add_latency*2+bram_latency+conv_latency  dbl_ovrd=off  reg_retiming=on  block_type=delay
  delay1 : xbsIndex_r4/Delay  en=off  latency=mult_latency+add_latency*2+bram_latency+conv_latency  dbl_ovrd=off  reg_retiming=on  block_type=delay
  delay2 : xbsIndex_r4/Delay  en=off  latency=mult_latency+add_latency*2+bram_latency+conv_latency  dbl_ovrd=off  reg_retiming=on  block_type=delay
  a_re : Outport  OutDataType=sfix(16)  OutScaling=2^0
  a_im : Outport  Port=2  OutDataType=sfix(16)  OutScaling=2^0
  bw_re : Outport  Port=3  OutDataType=sfix(16)  OutScaling=2^0
  bw_im : Outport  Port=4  OutDataType=sfix(16)  OutScaling=2^0
  sync_out : Outport  Port=5  OutDataType=sfix(16)  OutScaling=2^0
  wires:
  delay2/1 -> sync_out/1
  delay1/1 -> c_to_ri1/1
  delay0/1 -> c_to_ri/1
  a/1 -> delay0/1
  sync/1 -> delay2/1
  b/1 -> delay1/1
  c_to_ri/1 -> a_re/1
  c_to_ri/2 -> a_im/1
  c_to_ri1/1 -> bw_re/1
  c_to_ri1/2 -> bw_im/1

== system fft_direct_test/fft_direct/butterfly2_0/convert_of1 ==
  din : Inport  OutDataType=sfix(16)  OutScaling=2^0
  all_0s : xbsIndex_r4/Logical  logical_function=NAND  inputs=2  en=off  latency=latency  precision=Full  arith_type=Unsigned  n_bits=16  bin_pt=0  align_bp=on  dbl_ovrd=off  block_type=logical
  all_1s : xbsIndex_r4/Logical  logical_function=NAND  inputs=2  en=off  latency=latency  precision=Full  arith_type=Unsigned  n_bits=16  bin_pt=0  align_bp=on  dbl_ovrd=off  block_type=logical
  and : xbsIndex_r4/Logical  logical_function=AND  inputs=2  en=off  latency=0  precision=Full  arith_type=Unsigned  n_bits=16  bin_pt=0  align_bp=on  dbl_ovrd=off  block_type=logical
  convert : xbsIndex_r4/Convert  arith_type="Signed  (2's comp)"  n_bits=bit_width_o  bin_pt=binary_point_o  quantization=Truncate  overflow=Saturate  latency=latency  dbl_ovrd=off  pipeline=on  block_type=convert
      settings: block_version=10.1.1
  invert1 : xbsIndex_r4/Inverter  en=off  latency=0  dbl_ovrd=off  block_type=inv
  invert2 : xbsIndex_r4/Inverter  en=off  latency=0  dbl_ovrd=off  block_type=inv
  slice1 : xbsIndex_r4/Slice  nbits=1  boolean_output=on  mode=Upper Bit Location + Width  bit1=0  base1=MSB of Input  bit0=0  base0=LSB of Input  dbl_ovrd=off  block_type=slice
      settings: infoedit="Extracts a given range of bits from each input sample and presents it at the output.  The output type is ordinarily unsigned with binary point at zero, but can be Boolean when the slice is one bit wide.<P><P>Hardware notes: In hardware this block costs nothing."  block_version=10.1.1
  slice2 : xbsIndex_r4/Slice  nbits=1  boolean_output=on  mode=Upper Bit Location + Width  bit1=-1  base1=MSB of Input  bit0=0  base0=LSB of Input  dbl_ovrd=off  block_type=slice
      settings: infoedit="Extracts a given range of bits from each input sample and presents it at the output.  The output type is ordinarily unsigned with binary point at zero, but can be Boolean when the slice is one bit wide.<P><P>Hardware notes: In hardware this block costs nothing."  block_version=10.1.1
  dout : Outport
  of : Outport  Port=2
  wires:
  din/1 -> convert/1, slice1/1, slice2/1
  convert/1 -> dout/1
  slice1/1 -> all_1s/1, invert1/1
  invert1/1 -> all_0s/1
  slice2/1 -> all_1s/2, invert2/1
  invert2/1 -> all_0s/2
  all_0s/1 -> and/1
  all_1s/1 -> and/2
  and/1 -> of/1

== system fft_direct_test/fft_direct/butterfly2_0/convert_of2 ==
  din : Inport  OutDataType=sfix(16)  OutScaling=2^0
  all_0s : xbsIndex_r4/Logical  logical_function=NAND  inputs=2  en=off  latency=latency  precision=Full  arith_type=Unsigned  n_bits=16  bin_pt=0  align_bp=on  dbl_ovrd=off  block_type=logical
  all_1s : xbsIndex_r4/Logical  logical_function=NAND  inputs=2  en=off  latency=latency  precision=Full  arith_type=Unsigned  n_bits=16  bin_pt=0  align_bp=on  dbl_ovrd=off  block_type=logical
  and : xbsIndex_r4/Logical  logical_function=AND  inputs=2  en=off  latency=0  precision=Full  arith_type=Unsigned  n_bits=16  bin_pt=0  align_bp=on  dbl_ovrd=off  block_type=logical
  convert : xbsIndex_r4/Convert  arith_type="Signed  (2's comp)"  n_bits=bit_width_o  bin_pt=binary_point_o  quantization=Truncate  overflow=Saturate  latency=latency  dbl_ovrd=off  pipeline=on  block_type=convert
      settings: block_version=10.1.1
  invert1 : xbsIndex_r4/Inverter  en=off  latency=0  dbl_ovrd=off  block_type=inv
  invert2 : xbsIndex_r4/Inverter  en=off  latency=0  dbl_ovrd=off  block_type=inv
  slice1 : xbsIndex_r4/Slice  nbits=1  boolean_output=on  mode=Upper Bit Location + Width  bit1=0  base1=MSB of Input  bit0=0  base0=LSB of Input  dbl_ovrd=off  block_type=slice
      settings: infoedit="Extracts a given range of bits from each input sample and presents it at the output.  The output type is ordinarily unsigned with binary point at zero, but can be Boolean when the slice is one bit wide.<P><P>Hardware notes: In hardware this block costs nothing."  block_version=10.1.1
  slice2 : xbsIndex_r4/Slice  nbits=1  boolean_output=on  mode=Upper Bit Location + Width  bit1=-1  base1=MSB of Input  bit0=0  base0=LSB of Input  dbl_ovrd=off  block_type=slice
      settings: infoedit="Extracts a given range of bits from each input sample and presents it at the output.  The output type is ordinarily unsigned with binary point at zero, but can be Boolean when the slice is one bit wide.<P><P>Hardware notes: In hardware this block costs nothing."  block_version=10.1.1
  dout : Outport
  of : Outport  Port=2
  wires:
  din/1 -> convert/1, slice1/1, slice2/1
  convert/1 -> dout/1
  slice1/1 -> all_1s/1, invert1/1
  invert1/1 -> all_0s/1
  slice2/1 -> all_1s/2, invert2/1
  invert2/1 -> all_0s/2
  all_0s/1 -> and/1
  all_1s/1 -> and/2
  and/1 -> of/1

== system fft_direct_test/fft_direct/butterfly2_0/convert_of3 ==
  din : Inport  OutDataType=sfix(16)  OutScaling=2^0
  all_0s : xbsIndex_r4/Logical  logical_function=NAND  inputs=2  en=off  latency=latency  precision=Full  arith_type=Unsigned  n_bits=16  bin_pt=0  align_bp=on  dbl_ovrd=off  block_type=logical
  all_1s : xbsIndex_r4/Logical  logical_function=NAND  inputs=2  en=off  latency=latency  precision=Full  arith_type=Unsigned  n_bits=16  bin_pt=0  align_bp=on  dbl_ovrd=off  block_type=logical
  and : xbsIndex_r4/Logical  logical_function=AND  inputs=2  en=off  latency=0  precision=Full  arith_type=Unsigned  n_bits=16  bin_pt=0  align_bp=on  dbl_ovrd=off  block_type=logical
  convert : xbsIndex_r4/Convert  arith_type="Signed  (2's comp)"  n_bits=bit_width_o  bin_pt=binary_point_o  quantization=Truncate  overflow=Saturate  latency=latency  dbl_ovrd=off  pipeline=on  block_type=convert
      settings: block_version=10.1.1
  invert1 : xbsIndex_r4/Inverter  en=off  latency=0  dbl_ovrd=off  block_type=inv
  invert2 : xbsIndex_r4/Inverter  en=off  latency=0  dbl_ovrd=off  block_type=inv
  slice1 : xbsIndex_r4/Slice  nbits=1  boolean_output=on  mode=Upper Bit Location + Width  bit1=0  base1=MSB of Input  bit0=0  base0=LSB of Input  dbl_ovrd=off  block_type=slice
      settings: infoedit="Extracts a given range of bits from each input sample and presents it at the output.  The output type is ordinarily unsigned with binary point at zero, but can be Boolean when the slice is one bit wide.<P><P>Hardware notes: In hardware this block costs nothing."  block_version=10.1.1
  slice2 : xbsIndex_r4/Slice  nbits=1  boolean_output=on  mode=Upper Bit Location + Width  bit1=-1  base1=MSB of Input  bit0=0  base0=LSB of Input  dbl_ovrd=off  block_type=slice
      settings: infoedit="Extracts a given range of bits from each input sample and presents it at the output.  The output type is ordinarily unsigned with binary point at zero, but can be Boolean when the slice is one bit wide.<P><P>Hardware notes: In hardware this block costs nothing."  block_version=10.1.1
  dout : Outport
  of : Outport  Port=2
  wires:
  din/1 -> convert/1, slice1/1, slice2/1
  convert/1 -> dout/1
  slice1/1 -> all_1s/1, invert1/1
  invert1/1 -> all_0s/1
  slice2/1 -> all_1s/2, invert2/1
  invert2/1 -> all_0s/2
  all_0s/1 -> and/1
  all_1s/1 -> and/2
  and/1 -> of/1

== system fft_direct_test/fft_direct/butterfly2_0/convert_of4 ==
  din : Inport  OutDataType=sfix(16)  OutScaling=2^0
  all_0s : xbsIndex_r4/Logical  logical_function=NAND  inputs=2  en=off  latency=latency  precision=Full  arith_type=Unsigned  n_bits=16  bin_pt=0  align_bp=on  dbl_ovrd=off  block_type=logical
  all_1s : xbsIndex_r4/Logical  logical_function=NAND  inputs=2  en=off  latency=latency  precision=Full  arith_type=Unsigned  n_bits=16  bin_pt=0  align_bp=on  dbl_ovrd=off  block_type=logical
  and : xbsIndex_r4/Logical  logical_function=AND  inputs=2  en=off  latency=0  precision=Full  arith_type=Unsigned  n_bits=16  bin_pt=0  align_bp=on  dbl_ovrd=off  block_type=logical
  convert : xbsIndex_r4/Convert  arith_type="Signed  (2's comp)"  n_bits=bit_width_o  bin_pt=binary_point_o  quantization=Truncate  overflow=Saturate  latency=latency  dbl_ovrd=off  pipeline=on  block_type=convert
      settings: block_version=10.1.1
  invert1 : xbsIndex_r4/Inverter  en=off  latency=0  dbl_ovrd=off  block_type=inv
  invert2 : xbsIndex_r4/Inverter  en=off  latency=0  dbl_ovrd=off  block_type=inv
  slice1 : xbsIndex_r4/Slice  nbits=1  boolean_output=on  mode=Upper Bit Location + Width  bit1=0  base1=MSB of Input  bit0=0  base0=LSB of Input  dbl_ovrd=off  block_type=slice
      settings: infoedit="Extracts a given range of bits from each input sample and presents it at the output.  The output type is ordinarily unsigned with binary point at zero, but can be Boolean when the slice is one bit wide.<P><P>Hardware notes: In hardware this block costs nothing."  block_version=10.1.1
  slice2 : xbsIndex_r4/Slice  nbits=1  boolean_output=on  mode=Upper Bit Location + Width  bit1=-1  base1=MSB of Input  bit0=0  base0=LSB of Input  dbl_ovrd=off  block_type=slice
      settings: infoedit="Extracts a given range of bits from each input sample and presents it at the output.  The output type is ordinarily unsigned with binary point at zero, but can be Boolean when the slice is one bit wide.<P><P>Hardware notes: In hardware this block costs nothing."  block_version=10.1.1
  dout : Outport
  of : Outport  Port=2
  wires:
  din/1 -> convert/1, slice1/1, slice2/1
  convert/1 -> dout/1
  slice1/1 -> all_1s/1, invert1/1
  invert1/1 -> all_0s/1
  slice2/1 -> all_1s/2, invert2/1
  invert2/1 -> all_0s/2
  all_0s/1 -> and/1
  all_1s/1 -> and/2
  and/1 -> of/1
